simulink model "control_foc"  (R2025b)
settings: configuration reference "MCConfiguration" (kept outside this file)
libraries: mcbeeMathTransformLib x4, dspstat3 x2, slpidlib x2, simulink_extras x1, simulink x1
settings Model: DataDictionary=embeddedBoard_common.sldd  Creator=ascalzo  LastModifiedBy=rpumpo
settings ConfigSetRef: SourceName=MCConfiguration

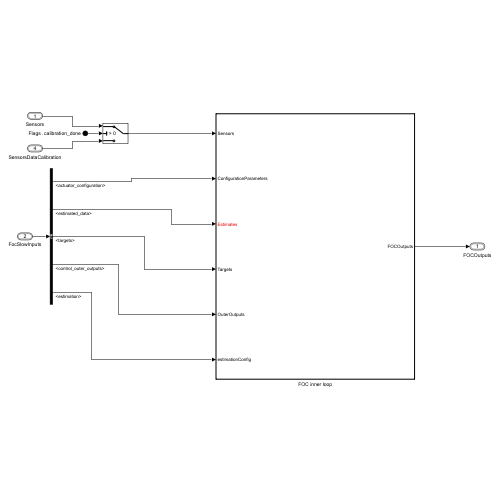
[thumbnail: Simulink's stored preview of the top-level diagram]
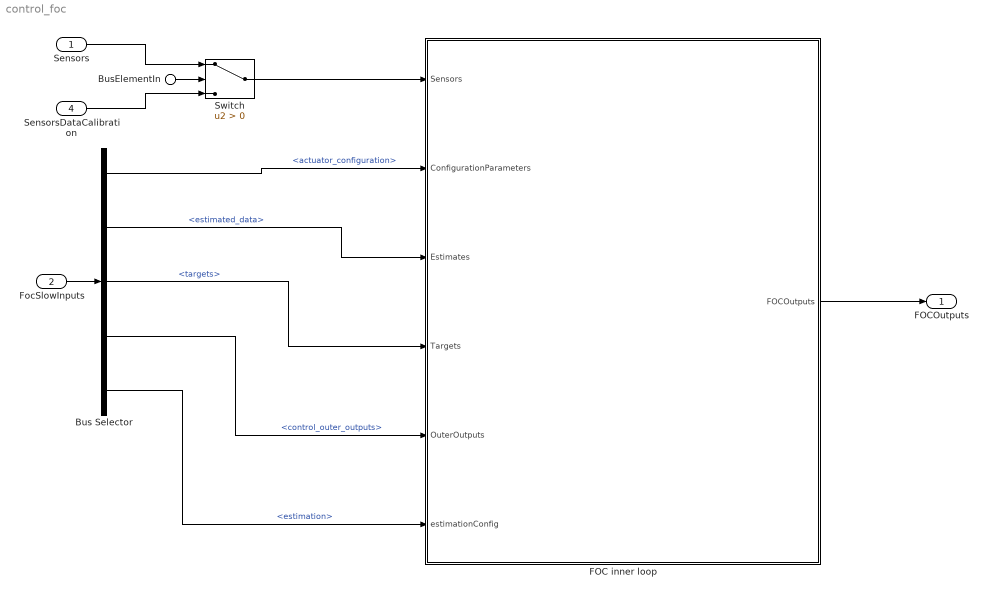
== system control_foc ==
  Sensors : Inport  OutDataTypeStr=Bus: SensorsData  BusOutputAsStruct=on
  FocSlowInputs : Inport  Port=2  OutDataTypeStr=Bus: FOCSlowInputs  BusOutputAsStruct=on
  BusElementIn : Inport  Port=3  PortName=Flags  Element=calibration_done
  SensorsDataCalibration : Inport  Port=4  OutDataTypeStr=Bus: SensorsData  BusOutputAsStruct=on
  Bus Selector : BusSelector  OutputSignals=actuator_configuration,estimated_data,targets,control_outer_outputs,global_configuration.estimation
  FOC inner loop : Subsystem  TreatAsAtomicUnit=on  RTWFcnName=FOCInnerLoop
      settings: RTWFcnNameOpts=User specified  RTWFileNameOpts=Use function name  FunctionInterfaceSpec=Allow arguments (Optimized)
  Switch : Switch  Criteria=u2 > Threshold  SaturateOnIntegerOverflow=off  InputSameDT=off
  FOCOutputs : Outport  OutDataTypeStr=Bus: FOCOutputs  BusOutputAsStruct=on
  wires:
  FOC inner loop/1(FOCOutputs) -> FOCOutputs/1
  Bus Selector/1 -> FOC inner loop/2(ConfigurationParameters)  "<actuator_configuration>"
  FocSlowInputs/1 -> Bus Selector/1
  Bus Selector/2 -> FOC inner loop/3(Estimates)  "<estimated_data>"
  Bus Selector/3 -> FOC inner loop/4(Targets)  "<targets>"
  Bus Selector/4 -> FOC inner loop/5(OuterOutputs)  "<control_outer_outputs>"
  Bus Selector/5 -> FOC inner loop/6(estimationConfig)  "<estimation>"
  BusElementIn/1 -> Switch/2
  Sensors/1 -> Switch/1
  SensorsDataCalibration/1 -> Switch/3
  Switch/1 -> FOC inner loop/1(Sensors)

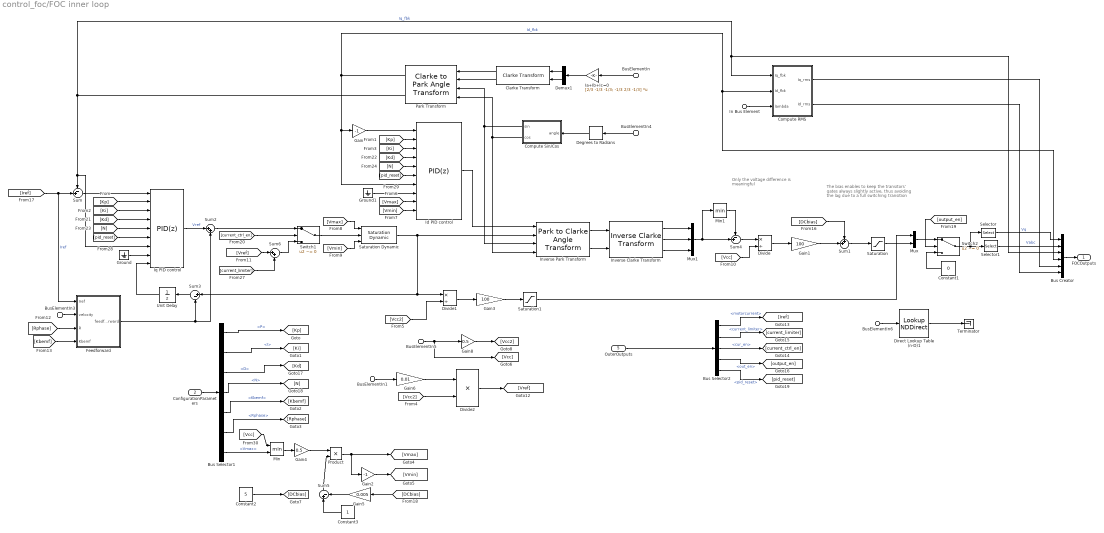
== system control_foc/FOC inner loop ==
  note: Only the voltage difference
      | is meaningful
  note: The bias enables to keep the transitors'
      | gates always slightly active, thus avoiding
      | the lag due to a full switching transition
  BusElementIn5 : Inport  Description=power supply voltage  PortName=Sensors  Element=driversensors.Vcc
  BusElementIn : Inport  PortName=Sensors  Element=motorsensors.Iabc
  BusElementIn4 : Inport  Description=electrical angle = angle * pole_pairs  PortName=Sensors  Element=motorsensors.electrical_angle
  BusElementIn6 : Inport  PortName=Sensors  Element=motorsensors.hallABC
  ConfigurationParameters : Inport  Port=2  OutDataTypeStr=Bus: ActuatorConfiguration
  BusElementIn3 : Inport  Description=Speed of the rotor BEFORE the reduction stage  Port=3  PortName=Estimates  Element=rotor_velocity
  BusElementIn1 : Inport  Port=4  PortName=Targets  Element=voltage
  OuterOutputs : Inport  Port=5  OutDataTypeStr=Bus: ControlOuterOutputs
  In Bus Element : Inport  Port=6  PortName=estimationConfig  Element=current_rms_lambda
  Bus Creator : BusCreator  Inputs=6  OutDataTypeStr=Bus: FOCOutputs  NonVirtualBus=on
      settings: InheritFromInputs=off
  Bus Selector1 : BusSelector  OutputSignals=pids.currentPID.P,pids.currentPID.I,pids.currentPID.D,pids.currentPID.N,motor.Kbemf,motor.Rphase,motor.Vmax
  Bus Selector2 : BusSelector  OutputSignals=motorcurrent,current_limiter,cur_en,out_en,pid_reset
  Clarke Transform : mcbeeMathTransformLib/Clarke Transform  VariantControl=Variant2  PowerInvariant=off  UseWithEmbedded=on  PhaseInput=Two inputs
      settings: LibrarySourceBlock=mcbcontrolslib/Clarke Transform
  Compute RMS : Subsystem  Variant=on  VariantControl=Subsystem
  Compute Sin/Cos : Subsystem  Variant=on  VariantControlMode=label  VariantControl=Compute Sin/Cos  LabelModeActiveChoice=Use standard library
  Constant1 : Constant  Value=0  OutDataTypeStr=single  SampleTime=-1
  Constant2 : Constant  Value=5  OutDataTypeStr=single  SampleTime=-1
  Constant3 : Constant  OutDataTypeStr=single  SampleTime=-1
  Degrees to Radians : simulink_extras/Transformations/Degrees to Radians
  Demux1 : Demux  Outputs=2
  Direct Lookup Table (n-D)1 : LookupNDDirect  NumberOfTableDimensions=1  Table=[-1,270,150,210,30,330,90,-1]  RemoveProtectionInput=on  TableDataTypeStr=single
  Divide : Product  Inputs=*/
  Divide1 : Product  Inputs=*/
  Divide2 : Product
  Feedforward : Subsystem  Variant=on  VariantControlMode=label  VariantControl=Subsystem  LabelModeActiveChoice=enabled
  Gain : Gain  Gain=-1
  Gain1 : Gain  Gain=100
  Gain2 : Gain  Gain=-1
  Gain3 : Gain  Gain=100
  Gain4 : Gain  Gain=0.5
  Gain5 : Gain  Gain=0.005
  Gain6 : Gain  Gain=0.01
  Gain8 : Gain  Gain=0.5
  Ground : Ground
  Ground1 : Ground
  Ia+Ib+Ic=0 : Gain  Gain=[2/3 -1/3 -1/3; -1/3 2/3 -1/3]  Multiplication=Matrix(K*u) (u vector)
  Id PID control : slpidlib/PID Controller  Controller=PID  Form=Parallel  TimeDomain=Discrete-time  UseExternalTs=off  SampleTime=-1  IntegratorMethod=Trapezoidal  FilterMethod=Trapezoidal  ControllerParametersSource=external  P=1  I=1  UseKiTs=off  D=0  UseExternalDerivativeSource=off  N=100  UseFilter=on  TunerSelectOption=Frequency Response Based  InitialConditionSource=external  InitialConditionForIntegrator=0  InitialConditionForFilter=0  DifferentiatorICPrevScaledInput=0  ExternalReset=rising  TrackingMode=off  Kt=1  LimitOutput=on  SatLimitsSource=external  UpperSaturationLimit=100  LowerSaturationLimit=-100  LinearizeAsGain=on  AntiWindupMode=clamping  Kb=1  LimitIntegrator=off  UpperIntegratorSaturationLimit=inf  LowerIntegratorSaturationLimit=-inf  POutMin=[]  POutMax=[]  IOutMin=[]  IOutMax=[]  DOutMin=[]  DOutMax=[]  NOutMin=[]  NOutMax=[]  SumOutMin=[]  SumOutMax=[]  SaturationOutMin=[]  SaturationOutMax=[]  PParamMin=[]  PParamMax=[]  IParamMin=[]  IParamMax=[]  DParamMin=[]  DParamMax=[]  NParamMin=[]  NParamMax=[]  KbParamMin=[]  KbParamMax=[]  KtParamMin=[]  KtParamMax=[]  KbOutMin=[]  KbOutMax=[]  KtOutMin=[]  KtOutMax=[]  IntegratorOutMin=[]  IntegratorOutMax=[]  FilterOutMin=[]  FilterOutMax=[]  SumI1OutMin=[]  SumI1OutMax=[]  SumI2OutMin=[]  SumI2OutMax=[]  SumI3OutMin=[]  SumI3OutMax=[]  SumI4OutMin=[]  SumI4OutMax=[]  SumDOutMin=[]  SumDOutMax=[]  DifferentiatorOutMin=[]  DifferentiatorOutMax=[]  FilterDiffOutCoefMin=[]  FilterDiffOutCoefMax=[]  ReciprocalOutMin=[]  ReciprocalOutMax=[]  SumDenOutMin=[]  SumDenOutMax=[]  SumNumOutMin=[]  SumNumOutMax=[]  DivideOutMin=[]  DivideOutMax=[]  UdiffTsProdOutMin=[]  UdiffTsProdOutMax=[]  NTsProdOutMin=[]  NTsProdOutMax=[]  UintegralTsProdOutMin=[]  UintegralTsProdOutMax=[]  UngainTsProdOutMin=[]  UngainTsProdOutMax=[]  ClampingZeroOutDataTypeStr=Inherit: Inherit via back propagation  ClampingZeroOutMin=[]  ClampingZeroOutMax=[]  FilterDenConstantOutDataTypeStr=Inherit: Inherit via back propagation  FilterDenConstantOutMin=[]  FilterDenConstantOutMax=[]  PCopyOutDataTypeStr=Inherit: Inherit via back propagation  PCopyOutMin=[]  PCopyOutMax=[]  NCopyOutDataTypeStr=Inherit: Inherit via back propagation  NCopyOutMin=[]  NCopyOutMax=[]  IntegratorContinuousStateAttributes=''  IntegratorStateMustResolveToSignalObject=off  IntegratorRTWStateStorageClass=Auto  FilterContinuousStateAttributes=''  FilterStateMustResolveToSignalObject=off  FilterRTWStateStorageClass=Auto  ParallelPVariant=ExternalParameters  IdealPVariant=Disabled  IVariant=ExternalParameters  DVariant=ExternalParameters  IntegratorVariant=Discrete  SatVariant=External  AWVariant=DiscClampingParallel  PCopyVariant=Disabled  TRVariant=Disabled  FdbkBlocksVariant=Feedback  IdealPFdbkVariant=Passthrough  SatFdbkVariant=Passthrough  DerivativeFilterVariant=TrapezoidalFilter  NVariant=ExternalParameters  NCopyVariant=ExternalParameters  FilterICVariant=ExternalICs  IntegratorICVariant=ExternalICs  ExternalResetVariant=ExternalReset  TRSumVariant=Passthrough  SumFdbkVariant=Enabled  SumVariant=Sum_PID  TsampFilterVariant=InternalTs  TsampNgainVariant=Passthrough  TsampIntegralVariant=Disabled_SignalSpec  ExternalSaturationOutDataTypeStr=Inherit: Same as second input  DerivativeSourceVariant=ErrorSignal  PreIntVariant=InternalPreInt
  Inverse Clarke Transform : mcbeeMathTransformLib/Inverse Clarke Transform  PowerInvariant=off  UseWithEmbedded=on  PhaseInput=Two inputs
      settings: LibrarySourceBlock=mcbcontrolslib/Inverse Clarke Transform
  Inverse Park Transform : mcbeeMathTransformLib/Park to Clarke Angle Transform  AxisAlignment=D-axis  UseWithEmbedded=on  PhaseInput=Two inputs  ThetaInput=Sine and Cosine electrical position  AngleInput=Per-unit  N_points=1024
      settings: LibrarySourceBlock=mcbcontrolslib/Inverse Park Transform
  Iq PID control : slpidlib/PID Controller  Controller=PID  Form=Parallel  TimeDomain=Discrete-time  UseExternalTs=off  SampleTime=-1  IntegratorMethod=Trapezoidal  FilterMethod=Trapezoidal  ControllerParametersSource=external  P=1  I=1  UseKiTs=off  D=0  UseExternalDerivativeSource=off  N=100  UseFilter=on  TunerSelectOption=Frequency Response Based  InitialConditionSource=external  InitialConditionForIntegrator=0  InitialConditionForFilter=0  DifferentiatorICPrevScaledInput=0  ExternalReset=rising  TrackingMode=on  Kt=1  LimitOutput=off  SatLimitsSource=internal  UpperSaturationLimit=100  LowerSaturationLimit=-100  LinearizeAsGain=on  AntiWindupMode=clamping  Kb=1  LimitIntegrator=off  UpperIntegratorSaturationLimit=inf  LowerIntegratorSaturationLimit=-inf  POutMin=[]  POutMax=[]  IOutMin=[]  IOutMax=[]  DOutMin=[]  DOutMax=[]  NOutMin=[]  NOutMax=[]  SumOutMin=[]  SumOutMax=[]  SaturationOutMin=[]  SaturationOutMax=[]  PParamMin=[]  PParamMax=[]  IParamMin=[]  IParamMax=[]  DParamMin=[]  DParamMax=[]  NParamMin=[]  NParamMax=[]  KbParamMin=[]  KbParamMax=[]  KtParamMin=[]  KtParamMax=[]  KbOutMin=[]  KbOutMax=[]  KtOutMin=[]  KtOutMax=[]  IntegratorOutMin=[]  IntegratorOutMax=[]  FilterOutMin=[]  FilterOutMax=[]  SumI1OutMin=[]  SumI1OutMax=[]  SumI2OutMin=[]  SumI2OutMax=[]  SumI3OutMin=[]  SumI3OutMax=[]  SumI4OutMin=[]  SumI4OutMax=[]  SumDOutMin=[]  SumDOutMax=[]  DifferentiatorOutMin=[]  DifferentiatorOutMax=[]  FilterDiffOutCoefMin=[]  FilterDiffOutCoefMax=[]  ReciprocalOutMin=[]  ReciprocalOutMax=[]  SumDenOutMin=[]  SumDenOutMax=[]  SumNumOutMin=[]  SumNumOutMax=[]  DivideOutMin=[]  DivideOutMax=[]  UdiffTsProdOutMin=[]  UdiffTsProdOutMax=[]  NTsProdOutMin=[]  NTsProdOutMax=[]  UintegralTsProdOutMin=[]  UintegralTsProdOutMax=[]  UngainTsProdOutMin=[]  UngainTsProdOutMax=[]  ClampingZeroOutDataTypeStr=Inherit: Inherit via back propagation  ClampingZeroOutMin=[]  ClampingZeroOutMax=[]  FilterDenConstantOutDataTypeStr=Inherit: Inherit via back propagation  FilterDenConstantOutMin=[]  FilterDenConstantOutMax=[]  PCopyOutDataTypeStr=Inherit: Inherit via back propagation  PCopyOutMin=[]  PCopyOutMax=[]  NCopyOutDataTypeStr=Inherit: Inherit via back propagation  NCopyOutMin=[]  NCopyOutMax=[]  IntegratorContinuousStateAttributes=''  IntegratorStateMustResolveToSignalObject=off  IntegratorRTWStateStorageClass=Auto  FilterContinuousStateAttributes=''  FilterStateMustResolveToSignalObject=off  FilterRTWStateStorageClass=Auto  ParallelPVariant=ExternalParameters  IdealPVariant=Disabled  IVariant=ExternalParameters  DVariant=ExternalParameters  IntegratorVariant=Discrete  SatVariant=Disabled  AWVariant=Passthrough  PCopyVariant=Disabled  TRVariant=Enabled  FdbkBlocksVariant=Feedback  IdealPFdbkVariant=Passthrough  SatFdbkVariant=Passthrough  DerivativeFilterVariant=TrapezoidalFilter  NVariant=ExternalParameters  NCopyVariant=ExternalParameters  FilterICVariant=ExternalICs  IntegratorICVariant=ExternalICs  ExternalResetVariant=ExternalReset  TRSumVariant=TrackingMode  SumFdbkVariant=Enabled  SumVariant=Sum_PID  TsampFilterVariant=InternalTs  TsampNgainVariant=Passthrough  TsampIntegralVariant=Disabled_SignalSpec  ExternalSaturationOutDataTypeStr=Inherit: Same as second input  DerivativeSourceVariant=ErrorSignal  PreIntVariant=InternalPreInt
  Min : MinMax  Inputs=2
  Min1 : MinMax
  Mux : Mux  Inputs=2
  Mux1 : Mux  Inputs=3
  Park Transform : mcbeeMathTransformLib/Clarke to Park Angle Transform  AxisAlignment=D-axis  UseWithEmbedded=on  PhaseInput=Two inputs  ThetaInput=Sine and Cosine electrical position  AngleInput=Per-unit  N_points=1024
      settings: LibrarySourceBlock=mcbcontrolslib/Park Transform
  Product : Product
  Saturation : Saturate  UpperLimit=100  LowerLimit=0
  Saturation Dynamic : simulink/Discontinuities/Saturation Dynamic  OutMin=[]  OutMax=[]  OutDataTypeStr=Inherit: Same as second input  OutDataType=fixdt(1, 16)  OutScaling=2^-10  DoSatur=off
  Saturation1 : Saturate  UpperLimit=100  LowerLimit=-100
  Selector : Selector  InputPortWidth=4  IndexOptions=Index vector (dialog)  Indices=1  OutputSizes=1
  Selector1 : Selector  InputPortWidth=4  IndexOptions=Index vector (dialog)  Indices=[2 3 4]  OutputSizes=1
  Sum : Sum  Inputs=-+|
  Sum1 : Sum  Inputs=++|
  Sum2 : Sum  Inputs=|++
  Sum3 : Sum  Inputs=|+-
  Sum4 : Sum  Inputs=-+|
  Sum5 : Sum  Inputs=|+-
  Sum6 : Sum  Inputs=|++
  Switch1 : Switch  Criteria=u2 ~= 0  SaturateOnIntegerOverflow=off  InputSameDT=off
  Switch2 : Switch  Criteria=u2 ~= 0  SaturateOnIntegerOverflow=off  InputSameDT=off
  Terminator : Terminator
  Unit Delay : UnitDelay  SampleTime=-1  HasFrameUpgradeWarning=on
  FOCOutputs : Outport  OutDataTypeStr=Bus: FOCOutputs
  wires:
  Sum/1 -> Iq PID control/1
  [current_ctrl_en] -> Switch1/2
  Park Transform/1 -> Id PID control/7, Gain/1, Compute RMS/2(Id_fbk), Bus Creator/4  "Id_fbk"
  Gain/1 -> Id PID control/1
  Park Transform/2 -> Iq PID control/7, Sum/1, Compute RMS/1(Iq_fbk), Bus Creator/3  "Iq_fbk"
  [Kp] -> Iq PID control/2
  [Ki] -> Iq PID control/3
  [Kp] -> Id PID control/2
  [Ki] -> Id PID control/3
  Constant1/1 -> Switch2/3
  Clarke Transform/1 -> Park Transform/1
  Clarke Transform/2 -> Park Transform/2
  Compute Sin/Cos/1(sin) -> Park Transform/3, Inverse Park Transform/3
  Inverse Clarke Transform/1 -> Mux1/1
  Inverse Clarke Transform/2 -> Mux1/2
  Inverse Clarke Transform/3 -> Mux1/3
  Inverse Park Transform/1 -> Inverse Clarke Transform/1
  Inverse Park Transform/2 -> Inverse Clarke Transform/2
  Id PID control/1 -> Inverse Park Transform/1
  Compute Sin/Cos/2(cos) -> Inverse Park Transform/4, Park Transform/4
  [Iref] -> Sum/2, Feedforward/1(Iref)  "Iref"
  Iq PID control/1 -> Sum2/1  "Vref"
  Sum3/1 -> Unit Delay/1
  Unit Delay/1 -> Iq PID control/9
  [Vmax] -> Id PID control/9
  [Vmin] -> Id PID control/10
  [Vmax] -> Saturation Dynamic/1
  [Vmin] -> Saturation Dynamic/3
  Divide/1 -> Gain1/1
  [Vcc] -> Divide/2
  Ia+Ib+Ic=0/1 -> Demux1/1
  Demux1/1 -> Clarke Transform/1
  Demux1/2 -> Clarke Transform/2
  Degrees to Radians/1 -> Compute Sin/Cos/1(angle)
  BusElementIn4/1 -> Degrees to Radians/1
  Bus Creator/1 -> FOCOutputs/1
  ConfigurationParameters/1 -> Bus Selector1/1
  [output_en] -> Switch2/2
  BusElementIn6/1 -> Direct Lookup Table (n-D)1/1
  Direct Lookup Table (n-D)1/1 -> Terminator/1
  [Kd] -> Iq PID control/4
  [Kd] -> Id PID control/4
  [N] -> Iq PID control/5
  [N] -> Id PID control/5
  Sum2/1 -> Switch1/1
  Switch1/1 -> Saturation Dynamic/2
  Saturation Dynamic/1 -> Sum3/1, Divide1/1, Inverse Park Transform/2
  Divide1/1 -> Gain3/1
  Gain3/1 -> Saturation1/1
  Sum1/1 -> Saturation/1
  Gain1/1 -> Sum1/2
  [DCbias] -> Sum1/1
  Min/1 -> Gain4/1
  Gain4/1 -> Product/1
  Sum4/1 -> Divide/1
  Mux1/1 -> Min1/1, Sum4/2
  Min1/1 -> Sum4/1
  Constant2/1 -> [DCbias]
  [DCbias] -> Gain5/1
  Product/1 -> Gain2/1, [Vmax]
  Gain2/1 -> [Vmin]
  Sum5/1 -> Product/2
  Constant3/1 -> Sum5/1
  Gain5/1 -> Sum5/2
  Sum6/1 -> Switch1/3
  [Vref] -> Sum6/1
  [current_limiter] -> Sum6/2
  Saturation/1 -> Mux/2
  Saturation1/1 -> Mux/1
  Mux/1 -> Switch2/1
  Switch2/1 -> Selector/1, Selector1/1
  Selector/1 -> Bus Creator/1  "Vq"
  Selector1/1 -> Bus Creator/2  "Vabc"
  [pid_reset] -> Iq PID control/6
  [pid_reset] -> Id PID control/6
  Compute RMS/1(Iq_rms) -> Bus Creator/5
  Compute RMS/2(Id_rms) -> Bus Creator/6
  In Bus Element/1 -> Compute RMS/3(lambda)
  OuterOutputs/1 -> Bus Selector2/1
  BusElementIn1/1 -> Gain6/1
  Divide2/1 -> [Vref]
  Bus Selector2/1 -> [Iref]  "<motorcurrent>"
  Bus Selector2/2 -> [current_limiter]  "<current_limiter>"
  Bus Selector2/3 -> [current_ctrl_en]  "<cur_en>"
  Bus Selector2/4 -> [output_en]  "<out_en>"
  Bus Selector2/5 -> [pid_reset]  "<pid_reset>"
  Bus Selector1/7 -> Min/2  "<Vmax>"
  Bus Selector1/6 -> [Rphase]  "<Rphase>"
  Bus Selector1/5 -> [Kbemf]  "<Kbemf>"
  Bus Selector1/4 -> [N]  "<N>"
  Bus Selector1/3 -> [Kd]  "<D>"
  Bus Selector1/2 -> [Ki]  "<I>"
  Bus Selector1/1 -> [Kp]  "<P>"
  BusElementIn5/1 -> Gain8/1, [Vcc]
  [Vcc] -> Min/1
  Ground/1 -> Iq PID control/8
  Ground1/1 -> Id PID control/8
  BusElementIn3/1 -> Feedforward/2(velocity)
  Feedforward/1(feedforward) -> Sum2/2, Sum3/2
  [Vcc2] -> Divide1/2
  Gain6/1 -> Divide2/1
  Gain8/1 -> [Vcc2]
  [Vcc2] -> Divide2/2
  [Rphase] -> Feedforward/3(R)
  [Kbemf] -> Feedforward/4(Kbemf)
  BusElementIn/1 -> Ia+Ib+Ic=0/1

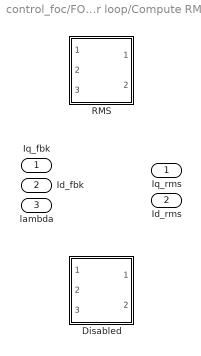
== system control_foc/FOC inner loop/Compute RMS ==
  Iq_fbk : Inport
  Id_fbk : Inport  Port=2
  lambda : Inport  Port=3
  Disabled : Subsystem  VariantControl=Temperature_estimation_switch == false
  RMS : Subsystem  VariantControl=Temperature_estimation_switch == true
  Iq_rms : Outport
  Id_rms : Outport  Port=2

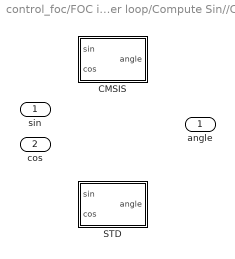
== system control_foc/FOC inner loop/Compute Sin//Cos ==
  angle : Inport
  CMSIS : Subsystem  VariantControl=Use look-up table
  STD : Subsystem  VariantControl=Use standard library
  sin : Outport
  cos : Outport  Port=2

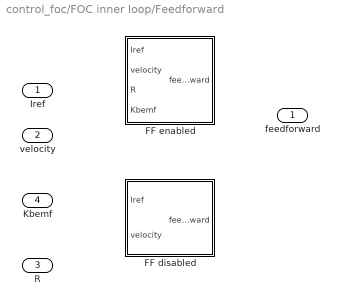
== system control_foc/FOC inner loop/Feedforward ==
  Iref : Inport
  velocity : Inport  Port=2
  R : Inport  Port=3
  Kbemf : Inport  Port=4
  FF disabled : Subsystem  VariantControl=disabled
  FF enabled : Subsystem  VariantControl=enabled
  feedforward : Outport

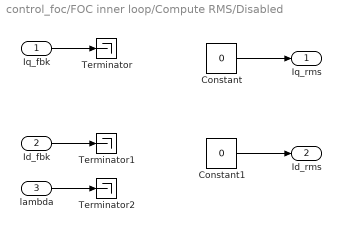
== system control_foc/FOC inner loop/Compute RMS/Disabled ==
  Iq_fbk : Inport
  Id_fbk : Inport  Port=2
  lambda : Inport  Port=3
  Constant : Constant  Value=0  OutDataTypeStr=single
  Constant1 : Constant  Value=0  OutDataTypeStr=single
  Terminator : Terminator
  Terminator1 : Terminator
  Terminator2 : Terminator
  Iq_rms : Outport
  Id_rms : Outport  Port=2
  wires:
  Constant/1 -> Iq_rms/1
  Constant1/1 -> Id_rms/1
  Iq_fbk/1 -> Terminator/1
  Id_fbk/1 -> Terminator1/1
  lambda/1 -> Terminator2/1

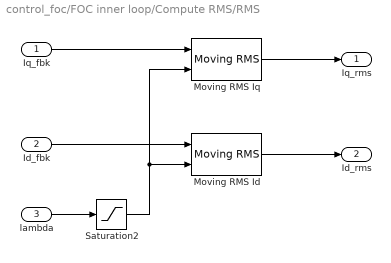
== system control_foc/FOC inner loop/Compute RMS/RMS ==
  Iq_fbk : Inport
  Id_fbk : Inport  Port=2
  lambda : Inport  Port=3
  Moving RMS Id : dspstat3/Moving RMS  Method=Exponential weighting  ForgettingFactorPort=on  SpecifyWindowLength=on  WindowLength=4  OverlapLength=3  AllowArbitraryInputLength=off  ForgettingFactor=1  SimulateUsing=Code generation
  Moving RMS Iq : dspstat3/Moving RMS  Method=Exponential weighting  ForgettingFactorPort=on  SpecifyWindowLength=on  WindowLength=4  OverlapLength=3  AllowArbitraryInputLength=off  ForgettingFactor=1  SimulateUsing=Code generation
  Saturation2 : Saturate  UpperLimit=1  LowerLimit=0
  Iq_rms : Outport
  Id_rms : Outport  Port=2
  wires:
  lambda/1 -> Saturation2/1
  Moving RMS Id/1 -> Id_rms/1
  Id_fbk/1 -> Moving RMS Id/1
  Iq_fbk/1 -> Moving RMS Iq/1
  Moving RMS Iq/1 -> Iq_rms/1
  Saturation2/1 -> Moving RMS Iq/2, Moving RMS Id/2

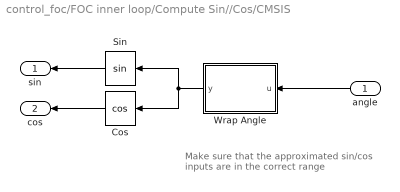
== system control_foc/FOC inner loop/Compute Sin//Cos/CMSIS ==
  note: Make sure that the approximated sin/cos
      | inputs are in the correct range
  angle : Inport
  Cos : Trigonometry  Operator=cos  ApproximationMethod=Lookup  NumberOfDataPoints=512
  Sin : Trigonometry  ApproximationMethod=Lookup  NumberOfDataPoints=512
  Wrap Angle : MATLAB Function  TreatAsAtomicUnit=on
  sin : Outport
  cos : Outport  Port=2
  wires:
  Cos/1 -> cos/1
  Wrap Angle/1(y) -> Cos/1, Sin/1
  angle/1 -> Wrap Angle/1(u)
  Sin/1 -> sin/1

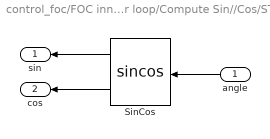
== system control_foc/FOC inner loop/Compute Sin//Cos/STD ==
  angle : Inport
  SinCos : Trigonometry  Operator=sincos
  sin : Outport
  cos : Outport  Port=2
  wires:
  SinCos/1 -> sin/1
  SinCos/2 -> cos/1
  angle/1 -> SinCos/1

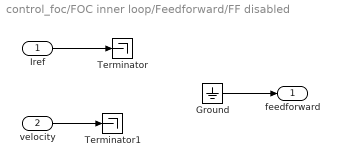
== system control_foc/FOC inner loop/Feedforward/FF disabled ==
  Iref : Inport
  velocity : Inport  Port=2
  Ground : Ground
  Terminator : Terminator
  Terminator1 : Terminator
  feedforward : Outport
  wires:
  Iref/1 -> Terminator/1
  velocity/1 -> Terminator1/1
  Ground/1 -> feedforward/1

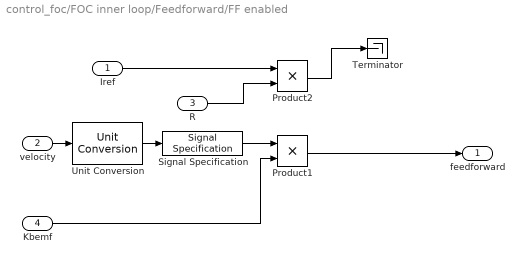
== system control_foc/FOC inner loop/Feedforward/FF enabled ==
  Iref : Inport
  velocity : Inport  Port=2
  R : Inport  Port=3
  Kbemf : Inport  Port=4
  Product1 : Product
  Product2 : Product
  Signal Specification : SignalSpecification  Unit=rad/s
  Terminator : Terminator
  Unit Conversion : UnitConversion
  feedforward : Outport
  wires:
  Product2/1 -> Terminator/1
  Kbemf/1 -> Product1/2
  R/1 -> Product2/2
  Product1/1 -> feedforward/1
  Iref/1 -> Product2/1
  velocity/1 -> Unit Conversion/1
  Unit Conversion/1 -> Signal Specification/1
  Signal Specification/1 -> Product1/1

== matlab function control_foc/FOC inner loop/Compute Sin//Cos/CMSIS/Wrap Angle ==
  data: u input; y output
function y = wrap_angle(u)

y = wrapTo2Pi(u);
